simulink model "EV_Truck_Model"  (R2022b)
settings: Solver=FixedStepAuto  StartTime=0  StopTime=26553  FixedStep=0.1  RelTol=1e-3
model workspace (MAT data in the model file):
  ADAS_MaxAccel = 2
  ADAS_MaxDecel = 2.5
  Adas_on_off = 0
  Batt_cap_ah = Simulink.Parameter
  Batt_cap_ah.Value = 180
  Batt_cap_ah.DataType = 'auto'
  Batt_cap_ah.Complexity = 'real'
  Batt_cap_ah.Dimensions = [1 1]
  Batt_rist_r0 = Simulink.Parameter
  Batt_rist_r0.Value = [0.5 0.5 0.5 0.5 0.5 0.5 0.5 0.5 0.5 0.5]
  Batt_rist_r0.DataType = 'auto'
  Batt_rist_r0.Complexity = 'real'
  Batt_rist_r0.Dimensions = [1 10]
  Batt_soc_s0 = Simulink.Parameter
  Batt_soc_s0.Value = [0 0.05 0.1 0.15 0.2 0.5 0.97 0.98 0.99 1]
  Batt_soc_s0.Description = 'Battery SOC WRT voltage v0'
  Batt_soc_s0.DataType = 'auto'
  Batt_soc_s0.Complexity = 'real'
  Batt_soc_s0.Dimensions = [1 10]
  Batt_volt_v0 = Simulink.Parameter
  Batt_volt_v0.Value = [2 2.5 2.8 3 3.1 3.2 3.3 3.32 3.4 3.65]
  Batt_volt_v0.Description = 'Battery Voltage WRT SOC value'
  Batt_volt_v0.DataType = 'auto'
  Batt_volt_v0.Complexity = 'real'
  Batt_volt_v0.Dimensions = [1 10]
  Motor_eff_100 = Simulink.Parameter
  Motor_eff_100.Value = [85  85  85  85  85  85  85  85  85  85  85; 85  85  85  85  85  85  85  85  85  85  85; 85  88  89  90  91  92  93  93  92  91  90; 85  86  88  90  91  94  94  93  91  90  90; 70  82  90  92  93  92  92  91  90  90  90; 78  82  90  91  90  89  89  89  89  89  89; 67  84  88  89  89  89  89  90  90  90  90; 68  82  85  89  89  89  89  89  89  89  89; 70  83  88  89  89  89  89  89  89  89  89; 71  84  89  89  89  89  89  89  89  89  89]
  Motor_eff_100.DataType = 'auto'
  Motor_eff_100.Complexity = 'real'
  Motor_eff_100.Dimensions = [10 11]
  Motor_eff_190 = Simulink.Parameter
  Motor_eff_190.Value = [55  60  65  67  68  69  85  83  77  72  68  67  65; 60  69  76  78  78  79  90  90  86  83  80  80  80; 65  73  79  82  83  84  93  93  91  89  88  86  85; 65  74  81  84  85  86  93  93  91  89  88  86  85; 65  75  83  85  87  87  93  94  93  91  90  90  85; 70  76  83  86  87  88  93  95  93  91  90  90  90; 70  76  84  87  88  89  94  95  93  92  91  90  90; 70  76  84  87  88  89  94  95  93  92  91  90  90; 70  76  84  87  89  90  94  95  94  93  91  90  90; 70  76  84  87  89  90  94  95  94  93  91  90  90; 70  76  84  87  89  90  94  95  94  93  91  90  90; 70  76  84  87  89  90  94  95  94  93  91  90  90; 65  75  84  87  89  90  94  95  94  92  90  90  90; 65  75  84  87  89  90  94  95  94  92  90  90  90; 65  75  84  87  89  90  94  95  93  91  90  90  90; 65  74  83  87  89  90  94  95  93  91  90  90  90; 65  74  83  87  89  90  94  94  93  91  90  90  90; 65  73  83  87  89  90  94  94  93  91  90  90  90; 65  73  83  86  88  90  94  94  92  91  90  90  90; 65  72  82  86  88  90  94  94  92  91  90  90  90; 65  72  82  86  88  90  94  94  92  91  90  90  90; 65  71  81  85  88  89  93  93  92  91  90  90  90; 65  71  81  86  88  89  93  92  92  91  90  90  90; 60  69  81  85  87  89  93  92  92  91  90  90  90; 60  68  80  85  87  89  93  92  92  91  90  90  90; 60  67  79  84  86  88  92  92  92  91  90  90  90; 60  66  78  83  86  88  92  92  92  91  90  90  90; 50  64  77  82  85  87  90  92  92  91  90  90  90; 50  63  76  82  84  86  90  92  92  91  90  90  90; 50  61  74  81  84  86  90  92  92  91  90  90  90; 50  62  74  80  83  86  90  92  92  91  90  90  90; 50  60  72  79  82  85  90  92  92  91  90  90  90]
  Motor_eff_190.DataType = 'auto'
  Motor_eff_190.Complexity = 'real'
  Motor_eff_190.Dimensions = [32 13]
  Motor_eff_95 = Simulink.Parameter
  Motor_eff_95.Value = [50 60 65 70 70 70 65 65 65 65 65 65 ... (598 elements, 23x26)]
  Motor_eff_95.DataType = 'auto'
  Motor_eff_95.Complexity = 'real'
  Motor_eff_95.Dimensions = [23 26]
  Motor_rpm_100 = Simulink.Parameter
  Motor_rpm_100.Value = [0; 900; 1100; 1300; 1500; 1800; 2000; 2500; 2700; 3000; 3200; 3500; 4000; 4500]
  Motor_rpm_100.DataType = 'auto'
  Motor_rpm_100.Complexity = 'real'
  Motor_rpm_100.Dimensions = [14 1]
  Motor_rpm_190 = Simulink.Parameter
  Motor_rpm_190.Value = [0 200 400 600 800 1000 1500 2000 2500 3000 3500 4000 4500]
  Motor_rpm_190.DataType = 'auto'
  Motor_rpm_190.Complexity = 'real'
  Motor_rpm_190.Dimensions = [1 13]
  Motor_rpm_95 = Simulink.Parameter
  Motor_rpm_95.Value = [0 180 360 540 720 900 1080 1260 1440 1620 1800 1980 2160 2340 2520 2700 2880 3060 3240 3420 3600 3780 3960 4140 4320 4500]
  Motor_rpm_95.DataType = 'auto'
  Motor_rpm_95.Complexity = 'real'
  Motor_rpm_95.Dimensions = [1 26]
  Motor_torque_pos_100 = Simulink.Parameter
  Motor_torque_pos_100.Value = [1000; 1000; 950; 900; 800; 700; 500; 425; 350; 300; 280; 260; 240; 220]
  Motor_torque_pos_100.DataType = 'auto'
  Motor_torque_pos_100.Complexity = 'real'
  Motor_torque_pos_100.Dimensions = [14 1]
  Motor_torque_pos_190 = Simulink.Parameter
  Motor_torque_pos_190.Value = [1417 1417 1417 1417 1417 1159 902 644 515 451 386 322 290]
  Motor_torque_pos_190.DataType = 'auto'
  Motor_torque_pos_190.Complexity = 'real'
  Motor_torque_pos_190.Dimensions = [1 13]
  Motor_torque_pos_95 = Simulink.Parameter
  Motor_torque_pos_95.Value = [611.111111111 611.111111111 611.111111111 611.111111111 611.111111111 611.111111111 611.111111111 611.111111111 611.111111111 555.555555556 527.777777778 472.222222222 416.666666667 388.888888889 361.111111111 333.333333333 305.555555556 277.777777778 250 250 222.222222222 222.222222222 194.444444444 194.444444444 194.444444444 194.444444444]
  Motor_torque_pos_95.DataType = 'auto'
  Motor_torque_pos_95.Complexity = 'real'
  Motor_torque_pos_95.Dimensions = [1 26]
  Motor_trq_190 = Simulink.Parameter
  Motor_trq_190.Value = [32; 64; 97; 129; 161; 193; 225; 258; 290; 322; 354; 386; 419; 451; 483; 515; 547; 580; 612; 644; 708; 773; 837; 902; 966; 1030; 1095; 1159; 1224; 1288; 1352; 1417]
  Motor_trq_190.DataType = 'auto'
  Motor_trq_190.Complexity = 'real'
  Motor_trq_190.Dimensions = [32 1]
  Motor_trq_95 = Simulink.Parameter
  Motor_trq_95.Value = [13.8888888889; 27.7777777778; 55.5555555556; 83.3333333333; 111.111111111; 138.888888889; 166.666666667; 194.444444444; 222.222222222; 250; 277.777777778; 305.555555556; 333.333333333; 361.111111111; 388.888888889; 416.666666667; 444.444444444; 472.222222222; 500; 527.777777778; 555.555555556; 583.333333333; 611.111111111]
  Motor_trq_95.DataType = 'auto'
  Motor_trq_95.Complexity = 'real'
  Motor_trq_95.Dimensions = [23 1]
  Sim_step = 0.1
  Test_DriveCycle = 0
  Trans_ratio = 6.142
  Veh_cog_fx = 1.69543
  Veh_cog_h = 0.605887
  Veh_cog_rx = 2.11956
  Veh_diff = 6.7
  Veh_whl_crr = 0.01
  Veh_whl_k = 180000
  Veh_whl_radius = 0.35
undefined symbols (not defined in the file): Batt_soc_init, canChannel, Elec_aux_sw, Elec_rgn_sw, Power_option, speed, time, Veh_mass
libraries: batteryecm_lib x170, simulink x14, canmsglib x9, canlib x7, autolibshared x5, nesl_utility x4, fl_lib x3, drivingvehiclecontroller x3, hdlsllib x3, sim3dlib x1, sim3dautolib x1, vrlib x1
(part 1 of 11)
settings Model: NumberOfSteps=5  SnapshotBufferSize=1000  PacingRate=0.100000  Creator=aprdc  LastModifiedBy=Ricky
settings OptimizationCC: DefaultParameterBehavior=Inlined  EnhancedBackFolding=on  PassReuseOutputArgsAs=Individual arguments  ZeroExternalMemoryAtStartup=off  ZeroInternalMemoryAtStartup=off  OptimizeBlockOrder=speed  DifferentSizesBufferReuse=on  OptimizationCustomize=off  EfficientTunableParamExpr=on
settings DebuggingCC: ParameterPrecisionLossMsg=none  ParameterTunabilityLossMsg=error
settings SFSimCC: MATLABDynamicMemAlloc=off
settings RTWCC: Description=Embedded Coder  SystemTargetFile=ert.tlc  TemplateMakefile=ert_default_tmf
settings CodeAppCC: ForceParamTrailComments=on  IgnoreCustomStorageClasses=off  OperatorAnnotations=on  SimulinkDataObjDesc=on  SFDataObjDesc=on  InsertBlockDesc=on
settings ERTTargetCC: TargetLangStandard=C99 (ISO)  GenerateSampleERTMain=on  InlinedParameterPlacement=NonHierarchical  ERTCustomFileTemplate=example_file_process.tlc

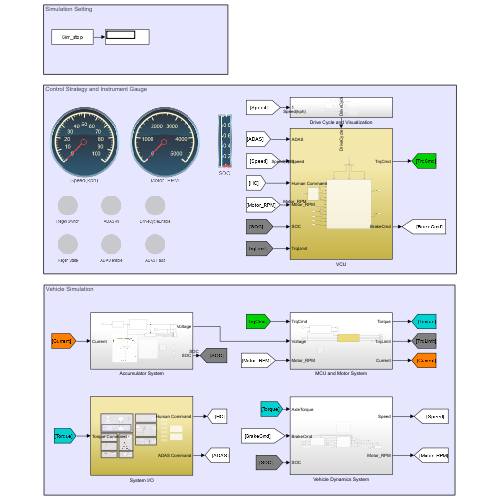
[thumbnail: Simulink's stored preview of the top-level diagram]
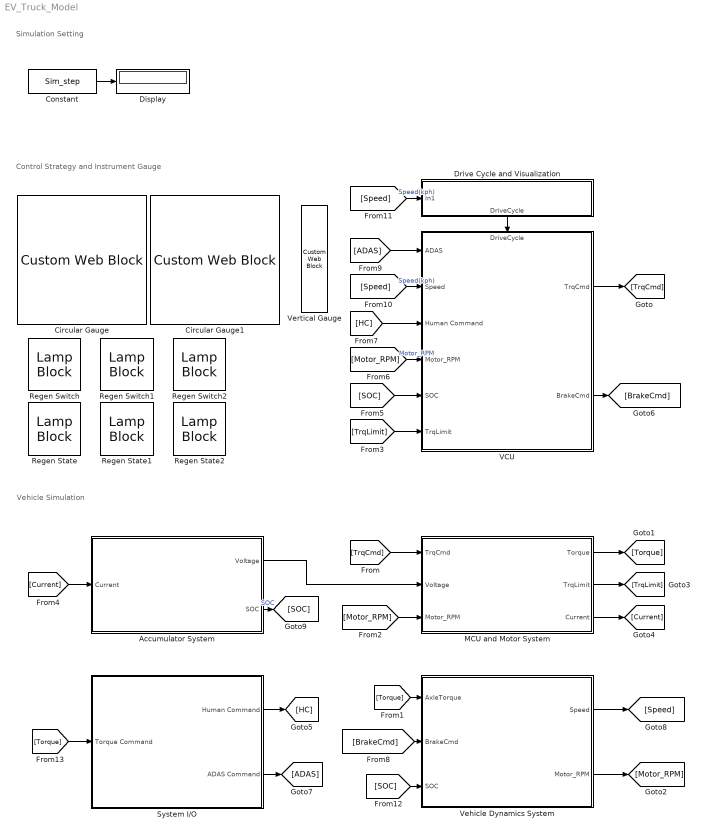
== system EV_Truck_Model ==
  note: Control Strategy and Instrument Gauge
  note: Vehicle Simulation
  note: Simulation Setting
  Accumulator System : Subsystem
  Circular Gauge : CustomWebBlock  LabelPosition=Bottom  ShowInitialText=on  Configuration="{\"components\":[{\"name\":\"CircularScaleComponent\",\"settings\":{\"bounds\":{\"max\":100,\"min\":0,\"tickInterval\":\"auto\"},\"direction\":\"cw\",\"flipLimits\":0,\"innerRadius\":0.75,\"internalTickHeightScaleFactor\":1,\"labelColor\":[255,255,200],\"labelFont\":{\"font\":\"Arial\",\"fontSize\":12},\"labelRadius\":0.528,\"labelTransparency\":1,\"minorTickHeightScaleFactor\":0.2,\"needleImage\":{\"size\":[200,50],\"src\":\"data:image\\/svg+xml;base64,PD94bWwgdmVyc2lvbj0iMS4wIiBlbmNvZGluZz0idXRmLTgiPz4KPCEtLSBHZW5lcmF0b3I6IEFkb2JlIElsbHVzdHJhdG9yIDI0LjEuMiwgU1ZHIEV4cG9ydCBQbHVnLUluIC4gU1ZHIFZlcnNpb246IDYuMDAgQnVpbGQgMCkgIC0tPgo8c3ZnIHZlcnNpb249IjEuMSIgaWQ9IkxheWVyXzEiIHhtbG5zPSJodHRwOi8vd3d3LnczLm9yZy8yMDAwL3N2ZyIgeG1sbnM6eGxpbms9Imh0dHA6Ly93d3cudzMub3JnLzE5OTkveGxpbmsiIHg9IjBweCIgeT0iMHB4IgoJIHZpZXdCb3g9IjAgMCAyMDAgNTAiIHN0eWxlPSJlbmFibGUtYmFja2dyb3VuZDpuZXcgMCAwIDIwMCA1MDsiIHhtbDpzcGFjZT0icHJlc2VydmUiPgo8c3R5bGUgdHlwZT0idGV4dC9jc3MiPgoJLnN0MHtmaWxsOiNFQzIxMjc7fQo8L3N0eWxlPgo8cGF0aCBjbGFzcz0ic3QwIiBkPSJNMTYyLjgsMTMuN0MxNjksNC40LDE4MS43LDEuOSwxOTEsOC4xczExLjgsMTguOSw1LjYsMjguMnMtMTguOSwxMS44LTI4LjIsNS42bDAsMAoJQzE1OS4xLDM1LjYsMTU2LjYsMjMsMTYyLjgsMTMuN0wxNjIuOCwxMy43eiBNMTY1LjgsMTUuOGMtNS4xLDcuNi0zLjEsMTcuOSw0LjYsMjNjNy42LDUuMSwxNy45LDMuMSwyMy00LjYKCWM1LjEtNy42LDMuMS0xNy45LTQuNi0yM2wwLDBDMTgxLjIsNi4yLDE3MC45LDguMiwxNjUuOCwxNS44eiIvPgo8cGF0aCBjbGFzcz0ic3QwIiBkPSJNMC40LDI1Ljl2LTMuM2wxNTktMi41Yy0wLjcsMi42LTAuNyw1LjIsMCw3LjhMMC40LDI1Ljl6Ii8+CjxjaXJjbGUgY2xhc3M9InN0MCIgY3g9IjE3OS42IiBjeT0iMjQiIHI9IjAuNyIvPgo8L3N2Zz4K\"},\"needleOffset\":[0.18464878250906522,0],\"needleOrientation\":-45,\"needleRotation\":180,\"needleSize\":{\"height\":0.11741692305346914,\"width\":0.46108337545091255},\"outerRadius\":0.9,\"position\":[0.05,0.05,0.9,0.9],\"referencePoint\":\"auto\",\"scaleAngle\":270,\"scaleAngleOffset\":135,\"scaleColors\":[],\"scaleColorsSize\":0.2,\"scaleDirection\":\"CW\",\"scalePosition\":[0,0,1,1],\"showLabels\":1,\"showMinorTicks\":1,\"showSpanLine\":1,\"showTicks\":1,\"tickColor\":[252,252,197],\"tickTransparency\":1,\"valueBarColor\":[0,114,189],\"valueBarPosition\":[0,0,1,1],\"valueBarSize\":0.2,\"valueBarTransparency\":1}},{\"name\":\"BackgroundImageComponent\",\"settings\":{\"image\":{\"size\":[500,500],\"src\":\"data:image\\/svg+xml;base64,PD94bWwgdmVyc2lvbj0iMS4wIiBlbmNvZGluZz0iVVRGLTgiIHN0YW5kYWxvbmU9Im5vIj8+CjxzdmcKICAgeG1sbnM6ZGM9Imh0dHA6Ly9wdXJsLm9yZy9kYy9lbGVtZW50cy8xLjEvIgogICB4bWxuczpjYz0iaHR0cDovL2NyZWF0aXZlY29tbW9ucy5vcmcvbnMjIgogICB4bWxuczpyZGY9Imh0dHA6Ly93d3cudzMub3JnLzE5OTkvMDIvMjItcmRmLXN5bnRheC1ucyMiCiAgIHhtbG5zOnN2Zz0iaHR0cDovL3d3dy53My5vcmcvMjAwMC9zdmciCiAgIHhtbG5zPSJodHRwOi8vd3d3LnczLm9yZy8yMDAwL3N2ZyIKICAgeG1sbnM6 ...(+9964 chars)\"},\"position\":[0,0,1,1],\"scaleMode\":\"0\"}},{\"name\":\"ForegroundImageComponent\",\"settings\":{\"image\":{\"size\":[0,0],\"src\":\"default\",\"srcOrientation\":[]},\"isForeground\":1,\"position\":[0,0,1,1],\"scaleMode\":\"0\"}}],\"settings\":{\"BindingType\":\"signal\",\"aspectRatio\":1.032258064516129,\"backgroundColor\":[0,0,0,\"1\"],\"backgroundOffset\":1,\"backgroundOpacity\":1,\"direction\":\"cw\",\"fixedAspectRatio\":\"on\",\"flipLimits\":0,\"orientation\":\"horizontal\",\"showBackgroundColor\":false,\"value\":0,\"version\":\"R2022b\"},\"type\":\"CircularGauge\"}"
  Circular Gauge1 : CustomWebBlock  LabelPosition=Bottom  ShowInitialText=on  Configuration="{\"components\":[{\"name\":\"CircularScaleComponent\",\"settings\":{\"bounds\":{\"max\":5000,\"min\":0,\"tickInterval\":\"auto\"},\"direction\":\"cw\",\"flipLimits\":0,\"innerRadius\":0.75,\"internalTickHeightScaleFactor\":1,\"labelColor\":[255,255,200],\"labelFont\":{\"font\":\"Arial\",\"fontSize\":12},\"labelRadius\":0.528,\"labelTransparency\":1,\"minorTickHeightScaleFactor\":0.2,\"needleImage\":{\"size\":[200,50],\"src\":\"data:image\\/svg+xml;base64,PD94bWwgdmVyc2lvbj0iMS4wIiBlbmNvZGluZz0idXRmLTgiPz4KPCEtLSBHZW5lcmF0b3I6IEFkb2JlIElsbHVzdHJhdG9yIDI0LjEuMiwgU1ZHIEV4cG9ydCBQbHVnLUluIC4gU1ZHIFZlcnNpb246IDYuMDAgQnVpbGQgMCkgIC0tPgo8c3ZnIHZlcnNpb249IjEuMSIgaWQ9IkxheWVyXzEiIHhtbG5zPSJodHRwOi8vd3d3LnczLm9yZy8yMDAwL3N2ZyIgeG1sbnM6eGxpbms9Imh0dHA6Ly93d3cudzMub3JnLzE5OTkveGxpbmsiIHg9IjBweCIgeT0iMHB4IgoJIHZpZXdCb3g9IjAgMCAyMDAgNTAiIHN0eWxlPSJlbmFibGUtYmFja2dyb3VuZDpuZXcgMCAwIDIwMCA1MDsiIHhtbDpzcGFjZT0icHJlc2VydmUiPgo8c3R5bGUgdHlwZT0idGV4dC9jc3MiPgoJLnN0MHtmaWxsOiNFQzIxMjc7fQo8L3N0eWxlPgo8cGF0aCBjbGFzcz0ic3QwIiBkPSJNMTYyLjgsMTMuN0MxNjksNC40LDE4MS43LDEuOSwxOTEsOC4xczExLjgsMTguOSw1LjYsMjguMnMtMTguOSwxMS44LTI4LjIsNS42bDAsMAoJQzE1OS4xLDM1LjYsMTU2LjYsMjMsMTYyLjgsMTMuN0wxNjIuOCwxMy43eiBNMTY1LjgsMTUuOGMtNS4xLDcuNi0zLjEsMTcuOSw0LjYsMjNjNy42LDUuMSwxNy45LDMuMSwyMy00LjYKCWM1LjEtNy42LDMuMS0xNy45LTQuNi0yM2wwLDBDMTgxLjIsNi4yLDE3MC45LDguMiwxNjUuOCwxNS44eiIvPgo8cGF0aCBjbGFzcz0ic3QwIiBkPSJNMC40LDI1Ljl2LTMuM2wxNTktMi41Yy0wLjcsMi42LTAuNyw1LjIsMCw3LjhMMC40LDI1Ljl6Ii8+CjxjaXJjbGUgY2xhc3M9InN0MCIgY3g9IjE3OS42IiBjeT0iMjQiIHI9IjAuNyIvPgo8L3N2Zz4K\"},\"needleOffset\":[0.18464878250906522,0],\"needleOrientation\":-45,\"needleRotation\":180,\"needleSize\":{\"height\":0.11741692305346914,\"width\":0.46108337545091255},\"outerRadius\":0.9,\"position\":[0.05,0.05,0.9,0.9],\"referencePoint\":\"auto\",\"scaleAngle\":270,\"scaleAngleOffset\":135,\"scaleColors\":[],\"scaleColorsSize\":0.2,\"scaleDirection\":\"CW\",\"scalePosition\":[0,0,1,1],\"showLabels\":1,\"showMinorTicks\":1,\"showSpanLine\":1,\"showTicks\":1,\"tickColor\":[252,252,197],\"tickTransparency\":1,\"valueBarColor\":[0,114,189],\"valueBarPosition\":[0,0,1,1],\"valueBarSize\":0.2,\"valueBarTransparency\":1}},{\"name\":\"BackgroundImageComponent\",\"settings\":{\"image\":{\"size\":[500,500],\"src\":\"data:image\\/svg+xml;base64,PD94bWwgdmVyc2lvbj0iMS4wIiBlbmNvZGluZz0iVVRGLTgiIHN0YW5kYWxvbmU9Im5vIj8+CjxzdmcKICAgeG1sbnM6ZGM9Imh0dHA6Ly9wdXJsLm9yZy9kYy9lbGVtZW50cy8xLjEvIgogICB4bWxuczpjYz0iaHR0cDovL2NyZWF0aXZlY29tbW9ucy5vcmcvbnMjIgogICB4bWxuczpyZGY9Imh0dHA6Ly93d3cudzMub3JnLzE5OTkvMDIvMjItcmRmLXN5bnRheC1ucyMiCiAgIHhtbG5zOnN2Zz0iaHR0cDovL3d3dy53My5vcmcvMjAwMC9zdmciCiAgIHhtbG5zPSJodHRwOi8vd3d3LnczLm9yZy8yMDAwL3N2ZyIKICAgeG1sbnM6 ...(+9964 chars)\"},\"position\":[0,0,1,1],\"scaleMode\":\"0\"}},{\"name\":\"ForegroundImageComponent\",\"settings\":{\"image\":{\"size\":[0,0],\"src\":\"default\",\"srcOrientation\":[]},\"isForeground\":1,\"position\":[0,0,1,1],\"scaleMode\":\"0\"}}],\"settings\":{\"BindingType\":\"signal\",\"aspectRatio\":1.032258064516129,\"backgroundColor\":[0,0,0,\"1\"],\"backgroundOffset\":1,\"backgroundOpacity\":1,\"direction\":\"cw\",\"fixedAspectRatio\":\"on\",\"flipLimits\":0,\"orientation\":\"horizontal\",\"showBackgroundColor\":false,\"value\":0,\"version\":\"R2022b\"},\"type\":\"CircularGauge\"}"
  Constant : Constant  Value=Sim_step
  Display : Display
  Drive Cycle and Visualization : Subsystem
      settings: PortSchema="{\"entries\":[{\"content\":{\"sides\":[{\"content\":{\"connectorIds\":[\"In1\"]},\"type\":\"ConnectorPlacement.EquallySpacedRectSide\",\"uuid\":\"15053575-2cbb-4954-870f-181623e09204\"},{\"content\":{\"connectorIds\":[],\"side\":\"RIGHT\"},\"type\":\"ConnectorPlacement.EquallySpacedRectSide\",\"uuid\":\"dfa9255f-4405-493c-ac30-8fbdd0eaef17\"},{\"content\":{\"connectorIds\":[],\"side\":\"TOP\"},\"type\":\"ConnectorPlacement.EquallySpacedRectSide\",\"uuid\":\"d91902c0-a975-413f-9369-a2252eb76ef9\"},{\"content\":{\"connectorIds\":[\"Out1\"],\"side\":\"BOTTOM\"},\"type\":\"ConnectorPlacement.EquallySpacedRectSide\",\"uuid\":\"f6469386-dded-411e-8143-94ee0ae8dca7\"}]},\"type\":\"ConnectorPlacement.EquallySpacedConnector\",\"uuid\":\"81b6e12d-61b2-488c-b50f-61c7eb1aaddd\"}],\"packageUris\":[\"http://schema.mathworks.com/mf0/Connector/R2020b\"],\"version\":\"1.0\"}"
  MCU and Motor System : Subsystem
  Regen State : LampBlock  LabelPosition=Bottom  Icon=Circle
  Regen State1 : LampBlock  LabelPosition=Bottom  Icon=Circle
  Regen State2 : LampBlock  LabelPosition=Bottom  Icon=Circle
  Regen Switch : LampBlock  LabelPosition=Bottom  Icon=Circle
  Regen Switch1 : LampBlock  LabelPosition=Bottom  Icon=Circle
  Regen Switch2 : LampBlock  LabelPosition=Bottom  Icon=Circle
  System I/O : Subsystem
  VCU : Subsystem
      settings: PortSchema="{\"entries\":[{\"content\":{\"sides\":[{\"content\":{\"connectorIds\":[\"In1\",\"In2\",\"In3\",\"In4\",\"In5\",\"In6\"]},\"type\":\"ConnectorPlacement.EquallySpacedRectSide\",\"uuid\":\"e23a74a3-5fad-4b77-90f0-abb788bacf61\"},{\"content\":{\"connectorIds\":[\"Out1\",\"Out2\"],\"side\":\"RIGHT\"},\"type\":\"ConnectorPlacement.EquallySpacedRectSide\",\"uuid\":\"a25eba40-4eae-44f7-8111-2c96fc21be99\"},{\"content\":{\"connectorIds\":[\"In7\"],\"side\":\"TOP\"},\"type\":\"ConnectorPlacement.EquallySpacedRectSide\",\"uuid\":\"5c32ab46-58dc-4220-8205-eddc509ab43c\"}]},\"type\":\"ConnectorPlacement.EquallySpacedConnector\",\"uuid\":\"b12ed4e3-c5a5-4aa5-b1ee-a92bdb93c66e\"}],\"packageUris\":[\"http://schema.mathworks.com/mf0/Connector/R2020b\"],\"version\":\"1.0\"}"
  Vehicle Dynamics System : Subsystem
  Vertical Gauge : CustomWebBlock  LabelPosition=Bottom  ShowInitialText=on  Configuration="{\"components\":[{\"name\":\"LinearScaleComponent\",\"settings\":{\"bounds\":{\"max\":1,\"min\":0,\"tickInterval\":\"auto\"},\"internalTickHeightScaleFactor\":0.5,\"labelColor\":[255,255,200],\"labelFont\":{\"font\":\"Arial\",\"fontSize\":12},\"labelOffset\":0.05,\"labelTransparency\":1,\"needleImage\":{\"size\":[21,75],\"src\":\"data:image\\/svg+xml;base64,PHN2ZyB4bWxucz0iaHR0cDovL3d3dy53My5vcmcvMjAwMC9zdmciIHhtbG5zOnhsaW5rPSJodHRwOi8vd3d3LnczLm9yZy8xOTk5L3hsaW5rIiB2aWV3Qm94PSIwIDAgMjEgNzUiPjxkZWZzPjxzdHlsZT4uY2xzLTF7ZmlsbDpub25lO30uY2xzLTJ7aXNvbGF0aW9uOmlzb2xhdGU7fS5jbHMtM3tjbGlwLXBhdGg6dXJsKCNjbGlwLXBhdGgpO30uY2xzLTR7b3BhY2l0eTowLjM7bWl4LWJsZW5kLW1vZGU6bXVsdGlwbHk7fS5jbHMtNXtmaWxsOiNlYjI2Mjk7fTwvc3R5bGU+PGNsaXBQYXRoIGlkPSJjbGlwLXBhdGgiIHRyYW5zZm9y ...(+1928 chars)\",\"srcOrientation\":\"horizontal\"},\"needleOffset\":[0.007413509060955519,0],\"needleSize\":{\"height\":0.11955094537815127,\"width\":0.7589285714285714},\"position\":[0.015821953781512604,0.06944444444444445,0.7996031746031746,0.9641544117647058],\"referencePoint\":\"auto\",\"scaleColors\":[{\"Color\":[0,114,189],\"Max\":0.5,\"Min\":0}],\"scaleColorsSize\":0.2,\"scaleDirection\":\"BT\",\"showLabels\":1,\"showMinorTicks\":0,\"showSpanLine\":1,\"showTicks\":1,\"tickColor\":[252,252,197],\"tickTransparency\":1,\"valueBarColor\":[23,89,176],\"valueBarOffset\":0,\"valueBarSize\":0.23,\"valueBarTransparency\":1}},{\"name\":\"BackgroundImageComponent\",\"settings\":{\"image\":{\"size\":[380,101],\"src\":\"data:image\\/svg+xml;base64,PHN2ZyBpZD0iZnJhbWUiIHhtbG5zPSJodHRwOi8vd3d3LnczLm9yZy8yMDAwL3N2ZyIgeG1sbnM6eGxpbms9Imh0dHA6Ly93d3cudzMub3JnLzE5OTkveGxpbmsiIHZpZXdCb3g9IjAgMCAzODAgMTAxIj48ZGVmcz48c3R5bGU+LmNscy0xe2ZpbGw6IzAwMmI0Mjt9LmNscy0ye2ZpbGw6IzQyNzA4Mjt9LmNscy0ze2ZpbGw6dXJsKCNyYWRpYWwtZ3JhZGllbnQpO308L3N0eWxlPjxyYWRpYWxHcmFkaWVudCBpZD0icmFkaWFsLWdyYWRpZW50IiBjeD0iMTkwIiBjeT0iNTAuNSIgcj0iMjY5LjIxIiBncmFkaWVudFVuaXRzPSJ1c2VyU3BhY2VPblVzZSI+PHN0b3Agb2Zmc2V0PSIwLjAxIiBzdG9wLWNvbG9yPSIjM2U0ZjU4Ii8+PHN0b3Agb2Zmc2V0PSIwLjA2IiBzdG9wLWNvbG9yPSIjNDQ1NzYxIi8+PHN0b3Agb2Zmc2V0PSIwLjE1IiBzdG9wLWNvbG9yPSIjNTU2YTc2Ii8+PHN0b3Agb2Zmc2V0PSIwLjI1IiBzdG9wLWNvbG9yPSIjNmQ4ODk1Ii8+PHN0b3Agb2Zmc2V0PSIwLjM4IiBzdG9wLWNvbG9yPSIjOGZiMmMzIi8+PHN0b3Agb2Zmc2V0PSIwLjUyIiBzdG9wLWNvbG9yPSIjYjZlNGZhIi8+PHN0b3Agb2Zmc2V0PSIxIiBzdG9wLWNvbG9yPSIjMTU0NjU3Ii8+PC9yYWRpYWxHcmFkaWVudD48L2RlZnM+PGcgaWQ9IkxheWVyXzIiIGRhdGEtbmFtZT0iTGF5ZXIgMiI+PGcgaWQ9IkxheWVyXzEtMiIgZGF0YS1uYW1lPSJMYXllciAxLTIiPjxyZWN0IGlkPSJyZWN0MTAzNiIgY2xhc3M9ImNscy0xIiB4PSIxMSIgeT0iMTEiIHdpZHRoPSIzNTgiIGhlaWdodD0iNzkiLz48cGF0aCBpZD0icGF0aDEwMzgiIGNsYXNzPSJjbHMtMiIgZD0iTTgsOFY5M0gzNzJWOFpNMzY5LDkwSDExVjExSDM2OVoiLz48cGF0aCBpZD0icGF0aDEwNDAiIGNsYXNzPSJjbHMtMyIgZD0iTTAsMFYxMDFIMzgwVjBaTTM3Miw5M0g4VjhIMzcyWiIvPjwvZz48L2c+PC9zdmc+\",\"srcOrientation\":\"horizontal\"},\"position\":[0,0,1,1],\"scaleMode\":\"0\"}},{\"name\":\"ForegroundImageComponent\",\"settings\":{\"image\":{\"size\":[0,0],\"src\":\"default\",\"srcOrientation\":[]},\"isForeground\":1,\"position\":[0,0,1,1],\"scaleMode\":\"0\"}}],\"settings\":{\"BindingType\":\"signal\",\"backgroundColor\":[0,0,0,\"1\"],\"backgroundOffset\":0,\"backgroundOpacity\":1,\"fixedAspectRatio\":\"on\",\"orientation\":\"vertical\",\"showBackgroundColor\":false,\"value\":0,\"version\":\"R2022b\"},\"type\":\"LinearGauge\"}"
  wires:
  [HC] -> VCU/3(Human Command)
  VCU/1(TrqCmd) -> [TrqCmd]
  [TrqCmd] -> MCU and Motor System/1(TrqCmd)
  MCU and Motor System/1(Torque) -> [Torque]
  [Torque] -> Vehicle Dynamics System/1(AxleTorque)
  [Motor_RPM] -> MCU and Motor System/3(Motor_RPM)
  Accumulator System/1(Voltage) -> MCU and Motor System/2(Voltage)
  MCU and Motor System/2(TrqLimit) -> [TrqLimit]
  [TrqLimit] -> VCU/6(TrqLimit)
  MCU and Motor System/3(Current) -> [Current]
  [Current] -> Accumulator System/1(Current)
  Vehicle Dynamics System/2(Motor_RPM) -> [Motor_RPM]
  [SOC] -> VCU/5(SOC)
  [Motor_RPM] -> VCU/4(Motor_RPM)  "Motor_RPM"
  System I/O/1(Human Command) -> [HC]
  VCU/2(BrakeCmd) -> [BrakeCmd]
  [BrakeCmd] -> Vehicle Dynamics System/2(BrakeCmd)
  System I/O/2(ADAS Command) -> [ADAS]
  Vehicle Dynamics System/1(Speed) -> [Speed]
  [Speed] -> VCU/2(Speed)  "Speed(kph)"
  [ADAS] -> VCU/1(ADAS)
  Accumulator System/2(SOC) -> [SOC]  "SOC"
  [Speed] -> Drive Cycle and Visualization/1(In1)  "Speed(kph)"
  Drive Cycle and Visualization/1(DriveCycle) -> VCU/7(DriveCycle)
  [SOC] -> Vehicle Dynamics System/3(SOC)
  [Torque] -> System I/O/1(Torque Command)
  Constant/1 -> Display/1
